simulink model "tc_static_v"  (R2026b)
settings: Solver=ode15s  StopTime=0.0015  MaxStep=1.9999999999999999e-07  RelTol=1e-06  AbsTol=1e-09
model workspace (MAT data in the model file):
  tcSweep = timeseries
  tcSweep.Name = 'unnamed'
  tcSweep.DataInfo = tsdata.datametadata
  tcSweep.DataInfo.Interpolation = tsdata.interpolation
  tcSweep.DataInfo.Interpolation.Fhandle : function handle (value not decoded)
  tcSweep.DataInfo.Interpolation.Name = 'linear'
  tcSweep.TimeInfo = tsdata.timemetadata
  tcSweep.TimeInfo.Length = 2
  tcSweep.TimeInfo.DuplicateTimes = 0
  tcSweep.TimeInfo.Time_ = [0; 0.0015]
  tcSweep.TimeInfo.Initialized = 1
  tcSweep.QualityInfo = tsdata.qualmetadata
  tcSweep.Data_ = [1; 1]
libraries: fl_lib x9, nesl_utility x6, ee_lib x1
settings Model: Creator=ganib  LastModifiedBy=ganib
settings SimscapeCC: SimscapeLogType=all  SimscapeNominalValues="[{\"value\":\"1\",\"unit\":\"A\"},{\"value\":\"1\",\"unit\":\"bar\"},{\"value\":\"1\",\"unit\":\"cm^2\"},{\"value\":\"1\",\"unit\":\"cm^3/s\"},{\"value\":\"1\",\"unit\":\"kJ/kg\"},{\"value\":\"1\",\"unit\":\"kW\"},{\"value\":\"1\",\"unit\":\"l\"},{\"value\":\"1\",\"unit\":\"N\"},{\"value\":\"1\",\"unit\":\"N*m\"},{\"value\":\"1\",\"unit\":\"V\"},{\"value\":\"0.001\",\"unit\":\"Wb\"}]"  SimscapeUseEnergyAccounting=off

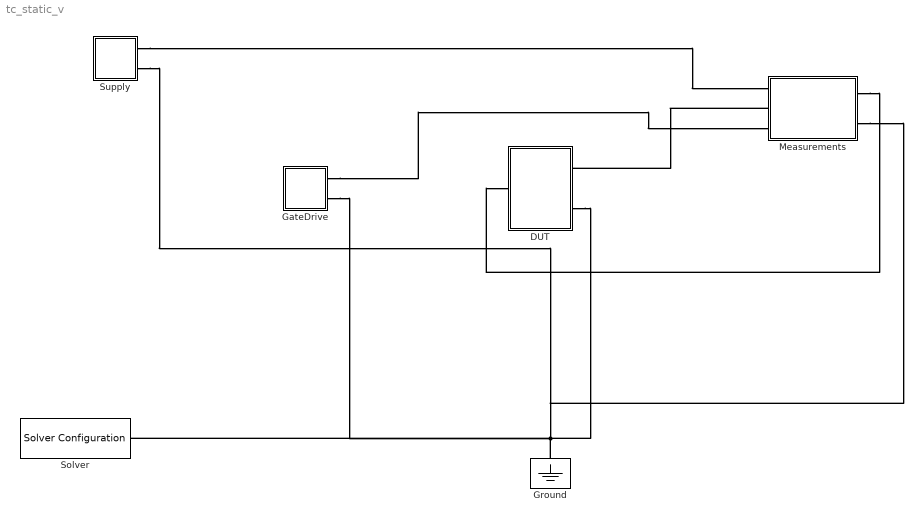
== system tc_static_v ==
  DUT : Subsystem
  GateDrive : Subsystem
  Ground : fl_lib/Electrical/Electrical Elements/Electrical Reference
  Measurements : Subsystem
  Solver : nesl_utility/Solver Configuration  PhysicalDomain=network_engine_domain  SubClassName=solver  LeftPortType=input  RightPortType=generic  Tones=[]  Harmonics=[]  SimulateNoise=off  Profile=off  UseLocalSampling=off  EnableSwitchedLinearOptims=on  FrequencyDomain=off  UseCCode=off  RelTol=0.001  AbsTol=0.001  MinStep=1e-09  ToWorkspace=off  RevertToSquareIcSolve=off  NumHomotopyIterations=100  PhasorMode=off  PhasorModeNumHarmonics=1  ConsistencySolver=NEWTON_XTOL_AFTER_FTOL  CanonicalOrdering=CANONICAL  OptimizeIntermediates=OPTIMIZED  MulticoreSolverChoice=BACKWARD_EULER  IndexReductionMethod=DerivativeReplacement  DoDC=on  ResidualTolerance=1e-09  ConsistencyTolSource=GLOBAL  ConsistencyAbsTol=0.001  ConsistencyRelTol=0.001  ConsistencyTolFactor=0.001  UseLocalSolver=off  LocalSolverChoice=NE_BACKWARD_EULER_ADVANCER  ResolveIndetEquations=on  FunctionEvalNumThread=1  LocalSolverSampleTime=0.001  DoFixedCost=off  MaxNonlinIter=3  MaxModeIter=2  ComputeImpulses=off  ImpulseIterations=2  LinearAlgebra=auto  LinearAlgebraNumThread=0  EquationFormulation=NE_TIME_EF  DelaysMemoryBudget=1024  AutomaticFiltering=on  FilteringTimeConstant=0.001  PartitionStorageMethod=AS_NEEDED  PartitionMemoryBudget=1024  PartitionMethod=BALANCED  MultibodyUseLocalSolver=off  MultibodyLocalSolverChoice=ODE1  MultibodyLocalSolverSampleTime=0.001
  Supply : Subsystem
  connections:
  DUT/RConn2 -- Ground/LConn1 -- Solver/RConn1 -- GateDrive/RConn2 -- Supply/RConn2 -- Measurements/RConn2
  Supply/RConn1 -- Measurements/LConn1
  Measurements/LConn2 -- DUT/RConn1
  GateDrive/RConn1 -- Measurements/LConn3
  Measurements/RConn1 -- DUT/LConn1

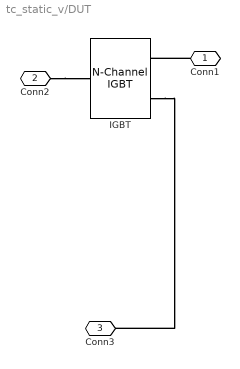
== system tc_static_v/DUT ==
  IGBT : ee_lib/Semiconductors & Converters/N-Channel IGBT  model_type=ee.enum.igbt.parameterization.equation  Ices=1.1501079949162614e-07 A  Vces=3300 V  Vth=6.3 V  Vce_sat=2.6 V  Ice_sat=1500 A  Vge_sat=15 V  Tmeas=25 degC  Vge_vec=[-1, 0, 2, 3, 5, 6, 7, 8, 10, 12, 15, 18, 20] V  Vce_vec=[0, .25, .5, .75, 1, 1.26, 1.51, 1.76, 2.01, 2.26, 2.51, 2.76, 3.01, 3.27, 3.52, 3.77, 4.02, 4.27, 4.52, 4.77] V  T_vec=[25, 125] degC  Ic_mat=[0, 0, 0, 0, 0, 0, 0, 0, 0, 0, 0, 0, 0, 0, 0, 0, 0, 0, 0, 0; 0, 0, 0, 0, 0, 0, 0, 0, 0, 0, 0, 0, 0, 0, 0, 0, 0, 0, 0, 0; 0, 0, 0, 0, 0, 0, 0, 0, 0, 0, 0, 0, 0, 0, 0, 0, 0, 0, 0, 0; 0, 0, 0, 0, 0, 0, 0, 0, 0, 0, 0, 0, 0, 0, 0, 0, 0, 0, 0, 0; 0, 0, 0, 0, 0, 0, 0, 0, 0, 0, 0, 0, 0, 0, 0, 0, 0, 0, 0, 0; 0, 0, 0, .81, 3.13, 4.97, 6.03, 6.53, 6.84, 7.01, 7.19, 7.32, 7.44, 7.55, 7.67, 7.78, 7.89, 8, 8.07, 8.07; 0, 0, 0, 1.07, 5.5, 12.93, 22.09, 29.14, 35.27, 38.97, 41.37, 43.08, 44.52, 45.45, 46.28, 46.85, 47.41, 47.76, 48.06, 48.36; 0, 0, 0, 1.1, 6.99, 16.51, 28.38, 41.53, 55.76, 69.08, 80.5, 89.56, 96.13, 101.45, 105.15, 107.99, 110.09, 111.87, 113.54, 114.95; 0, 0, 0, 1.36, 6.26, 17.43, 33.6, 50.43, 71.75, 93.61, 114.64, 134.42, 151.44, 164.25, 177.06, 189.88, 202.69, 215.51, 228.32, 241.14; 0, 0, 0, 1.42, 6.4, 18.7, 36.19, 55.23, 79.71, 106.22, 131.28, 156.62, 182.79, 208.97, 235.15, 261.32, 287.5, 313.67, 339.85, 366.02; 0, 0, 0, 1.45, 6.81, 20.01, 39.61, 60.63, 88.74, 117.7, 147.16, 191.87, 237.14, 282.42, 327.69, 372.96, 418.23, 463.5, 508.77, 554.04; 0, 0, 0, 1.49, 6.97, 20.55, 41.34, 64.15, 94.91, 126.1, 170.16, 233.77, 297.38, 360.98, 424.59, 488.19, 551.8, 615.4, 679.01, 742.62; 0, 0, 0, 1.5, 7.5, 20.96, 42.17, 66.19, 98.34, 131.14, 187.84, 263.46, 339.09, 414.72, 490.34, 565.97, 641.6, 717.22, 792.85, 868.48] A  Ic_mat_3D=zeros(13, 20, 2) A  C_param=ee.enum.igbt.capacitanceParam.fixedciss  C_GE=23.7 nF  C_GC=2.7 nF  C_CE=0 nF  C_ies=1.6400000000000001e-07 F  C_res=1.3999999999999999e-09 F  C_oes=1.0999999999999999e-08 F  C_GE_vec=[25, 31, 26.5, 24.9, 25, 24.9, 24.6, 24.7, 24.8] nF  C_GC_vec=[55, 9, 5.5, 3.1, 2.5, 2.1, 1.9, 1.8, 1.7] nF  C_Vge_vec=0 V  C_CE_vec=[5, 11, 6.5, 4.9, 3.5, 2.7, 2.1, 1.7, 1.4] nF  C_ies_vec=[80, 40, 32, 28, 27.5, 27, 26.5, 26.5, 26.5] nF  C_res_vec=[55, 9, 5.5, 3.1, 2.5, 2.1, 1.9, 1.8, 1.7] nF  C_oes_vec=[60, 20, 12, 8, 6, 4.8, 4, 3.5, 3.1] nF  C_Vce_vec=[0, 1, 2, 5, 10, 15, 20, 25, 30] V  charge_linearity_param=ee.enum.igbt.cgcLinearity.constant  C_OX=20 nF  V_C_OX=-5 V  TF=1.9999999999999999e-07 s  TT=0 us  LeadRc=0 Ohm  LeadRe=0 Ohm  LeadRg=0 Ohm  LC=0 nH  LE=0 nH  LG=0 nH  ec=1  VAF=200 V  RC=4.5e-05 Ohm  RE=4.5e-05 Ohm  RG=0.5 Ohm  BF=50  T_param=ee.enum.igbt.temperatureParameterization.IcesVce  Ices_T2=0.0040000000000000001 A  EG=1.11 eV  Vce_sat_T2=3.2 V  Tmeas2=125 degC  XTI=3  BEX=-1.5  RG_alpha=0 1/K  Tdevice=25 degC  Tdevice_3D=25 degC  ig_specify=off  ig_priority=None  ig=0 A  ig_nominal_specify=off  ig_nominal_value=1  ig_nominal_unit=A  ic_specify=off  ic_priority=None  ic=0 A  ic_nominal_specify=off  ic_nominal_value=1  ic_nominal_unit=A  vge_specify=off  vge_priority=None  vge=0 V  vge_nominal_specify=off  vge_nominal_value=1  vge_nominal_unit=V  vce_specify=off  vce_priority=None  vce=0 V  vce_nominal_specify=off  vce_nominal_value=1  vce_nominal_unit=V  v_Cge_specify=off  v_Cge_priority=High  v_Cge=0 V  v_Cge_nominal_specify=off  v_Cge_nominal_value=1  v_Cge_nominal_unit=V  v_Cce_specify=off  v_Cce_priority=High  v_Cce=0 V  v_Cce_nominal_specify=off  v_Cce_nominal_value=1  v_Cce_nominal_unit=V  thermal_network_parameterization=ee.enum.thermalNetworkTopology.junctionCase  Rth=[0, 10] K/W  Rth_Cauer=[1, 3, 10] K/W  Rth_Foster=[.08, .14, .22, .16] K/W  thermal_mass_parameterization=ee.enum.thermalNetwork.timeconstant  thermal_mass=[0, 1] J/K  thermal_mass_Cauer=[.1, .3, 1] J/K  thermal_mass_Foster=[.001, .005, .05, .5] J/K  thermal_time_constant=[0, 10] s  thermal_time_constant_Cauer=[1, 3, 10] s  thermal_time_constant_Foster=[7e-05, .0007, .01, .08] s  thermal_mass_initial_temperatures=[25, 25] degC  thermal_mass_initial_temperatures_Cauer=[25, 25, 25] degC  Tvec_initial_Foster=[25, 25, 25, 25] degC  Ic_vec1=[0, 10, 50, 100, 200, 400, 600] A  Vce_vec1=[0, 1.1, 1.3, 1.45, 1.75, 2.25, 2.7] V  Rmiller=0.1 Ohm  Goff=1e-5 1/Ohm  t_on=0.07 us  t_rise=0.7 us  t_off=0.2 us  t_fall=0.5 us  v_meas=300 V  vStartTurnOn_specify=off  vStartTurnOn_priority=None  vStartTurnOn=1 V  tStartTurnOn_specify=off  tStartTurnOn_priority=None  tStartTurnOn=0 s  vStartTurnOff_specify=off  vStartTurnOff_priority=None  vStartTurnOff=0.5 V  tStartTurnOff_specify=off  tStartTurnOff_priority=None  tStartTurnOff=0 s  Tj_vec1=[298.15, 398.15] K  Vce_mat1=[0, 1.1, 1.3, 1.45, 1.75, 2.25, 2.7; 0, 1, 1.15, 1.35, 1.7, 2.35, 3] V  Tj_vec_loss=[298.15, 398.15] K  Ic_vec_loss=[0, 10, 50, 100, 200, 400, 600] A  E_turn_on_mat1=[0, .2, 1, 2, 4, 8, 15; 0, .3, 1.3, 2.5, 5, 11, 18] * 1e-3 J  E_turn_off_mat1=[0, .3, 1.5, 3, 6, 15, 25; 0, .7, 3.3, 6.5, 13, 25, 35] * 1e-3 J  iStartTurnOff_specify=off  iStartTurnOff_priority=None  iStartTurnOff=0 A  Tdevice_specify=off  Tdevice_priority=None
  Conn1 : PMIOPort  Side=Right
  Conn2 : PMIOPort  Port=2  Side=Left
  Conn3 : PMIOPort  Port=3  Side=Right
  connections:
  Conn1/RConn1 -- IGBT/RConn1
  Conn2/RConn1 -- IGBT/LConn1
  IGBT/RConn2 -- Conn3/RConn1

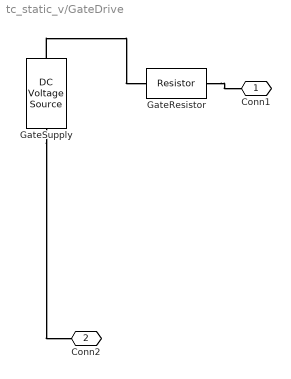
== system tc_static_v/GateDrive ==
  GateResistor : fl_lib/Electrical/Electrical Elements/Resistor  R=0 Ohm  i_specify=off  i_priority=None  i=0 A  i_nominal_specify=off  i_nominal_value=1  i_nominal_unit=A  v_specify=off  v_priority=None  v=0 V  v_nominal_specify=off  v_nominal_value=1  v_nominal_unit=V
  GateSupply : fl_lib/Electrical/Electrical Sources/DC Voltage Source  v0=15 V
  Conn1 : PMIOPort  Side=Right
  Conn2 : PMIOPort  Port=2  Side=Right
  connections:
  GateSupply/LConn1 -- GateResistor/LConn1
  GateResistor/RConn1 -- Conn1/RConn1
  GateSupply/RConn1 -- Conn2/RConn1

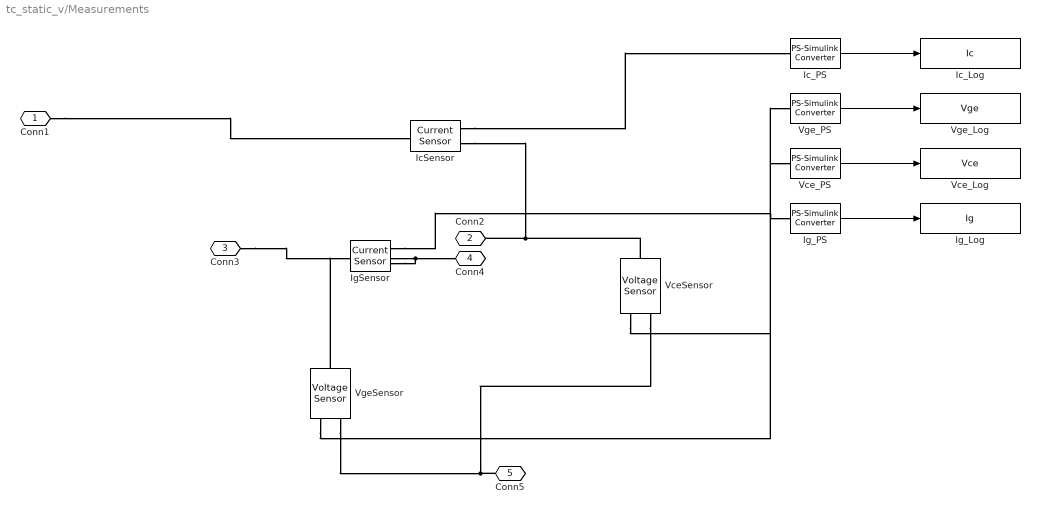
== system tc_static_v/Measurements ==
  IcSensor : fl_lib/Electrical/Electrical Sensors/Current Sensor
  Ic_Log : ToWorkspace  VariableName=Ic  SaveFormat=Timeseries  SampleTime=-1
  Ic_PS : nesl_utility/PS-Simulink Converter  PhysicalDomain=network_engine_domain  SubClassName=ps_output  LeftPortType=input  RightPortType=output  PseudoPeriodic=off  Frequencies=[]  VectorFormat=inherit  Unit=A  AffineConversion=off
  IgSensor : fl_lib/Electrical/Electrical Sensors/Current Sensor
  Ig_Log : ToWorkspace  VariableName=Ig  SaveFormat=Timeseries  SampleTime=-1
  Ig_PS : nesl_utility/PS-Simulink Converter  PhysicalDomain=network_engine_domain  SubClassName=ps_output  LeftPortType=input  RightPortType=output  PseudoPeriodic=off  Frequencies=[]  VectorFormat=inherit  Unit=A  AffineConversion=off
  VceSensor : fl_lib/Electrical/Electrical Sensors/Voltage Sensor
  Vce_Log : ToWorkspace  VariableName=Vce  SaveFormat=Timeseries  SampleTime=-1
  Vce_PS : nesl_utility/PS-Simulink Converter  PhysicalDomain=network_engine_domain  SubClassName=ps_output  LeftPortType=input  RightPortType=output  PseudoPeriodic=off  Frequencies=[]  VectorFormat=inherit  Unit=V  AffineConversion=off
  VgeSensor : fl_lib/Electrical/Electrical Sensors/Voltage Sensor
  Vge_Log : ToWorkspace  VariableName=Vge  SaveFormat=Timeseries  SampleTime=-1
  Vge_PS : nesl_utility/PS-Simulink Converter  PhysicalDomain=network_engine_domain  SubClassName=ps_output  LeftPortType=input  RightPortType=output  PseudoPeriodic=off  Frequencies=[]  VectorFormat=inherit  Unit=V  AffineConversion=off
  Conn1 : PMIOPort  Side=Left
  Conn2 : PMIOPort  Port=2  Side=Left
  Conn3 : PMIOPort  Port=3  Side=Left
  Conn4 : PMIOPort  Port=4  Side=Right
  Conn5 : PMIOPort  Port=5  Side=Right
  wires:
  Vce_PS/1 -> Vce_Log/1
  Ic_PS/1 -> Ic_Log/1
  Vge_PS/1 -> Vge_Log/1
  Ig_PS/1 -> Ig_Log/1
  connections:
  IcSensor/RConn1 -- Ic_PS/LConn1
  IgSensor/RConn1 -- Ig_PS/LConn1
  IcSensor/RConn2 -- Conn2/RConn1 -- VceSensor/LConn1
  VgeSensor/RConn1 -- Vge_PS/LConn1
  VgeSensor/LConn1 -- Conn4/RConn1 -- IgSensor/RConn2
  VceSensor/RConn1 -- Vce_PS/LConn1
  Conn3/RConn1 -- IgSensor/LConn1
  Conn1/RConn1 -- IcSensor/LConn1
  Conn5/RConn1 -- VceSensor/RConn2 -- VgeSensor/RConn2

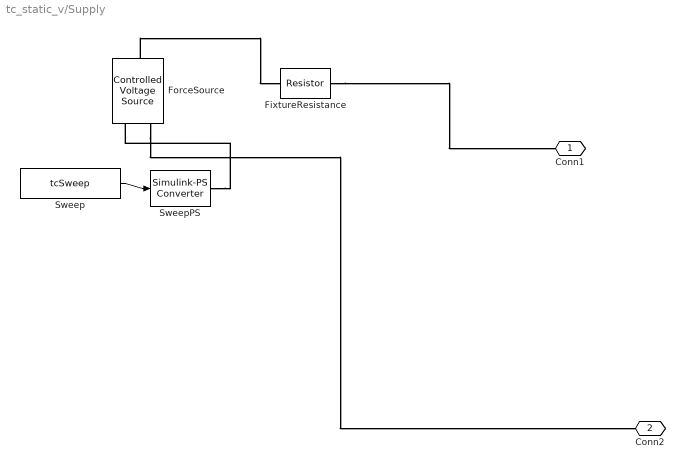
== system tc_static_v/Supply ==
  FixtureResistance : fl_lib/Electrical/Electrical Elements/Resistor  R=0.1 Ohm  i_specify=off  i_priority=None  i=0 A  i_nominal_specify=off  i_nominal_value=1  i_nominal_unit=A  v_specify=off  v_priority=None  v=0 V  v_nominal_specify=off  v_nominal_value=1  v_nominal_unit=V
  ForceSource : fl_lib/Electrical/Electrical Sources/Controlled Voltage Source
  Sweep : FromWorkspace  VariableName=tcSweep  Interpolate=off  OutputAfterFinalValue=Holding final value
  SweepPS : nesl_utility/Simulink-PS Converter  PhysicalDomain=network_engine_domain  SubClassName=ps_input  LeftPortType=input  RightPortType=output  PseudoPeriodic=off  Frequencies=[]  NoiseDistribution=none  NoiseParameters=[]  Unit=V  AffineConversion=off  FilteringAndDerivatives=filter  SimscapeFilterOrder=1  InputFilterTimeConstant=1e-6  UdotUserProvided=0
  Conn1 : PMIOPort  Side=Right
  Conn2 : PMIOPort  Port=2  Side=Right
  wires:
  Sweep/1 -> SweepPS/1
  connections:
  ForceSource/RConn2 -- Conn2/RConn1
  ForceSource/LConn1 -- FixtureResistance/LConn1
  SweepPS/RConn1 -- ForceSource/RConn1
  FixtureResistance/RConn1 -- Conn1/RConn1
